simulink model "emso3"  (Simulink 7.1)
settings: Solver=VariableStepDiscrete  StartTime=0.0  StopTime=5  RelTol=1e-3
settings Model: Creator=lades  LastModifiedBy=Administrator
settings DataIOCC: ExternalInput=Az
settings DebuggingCC: SolverPrmCheckMsg=none

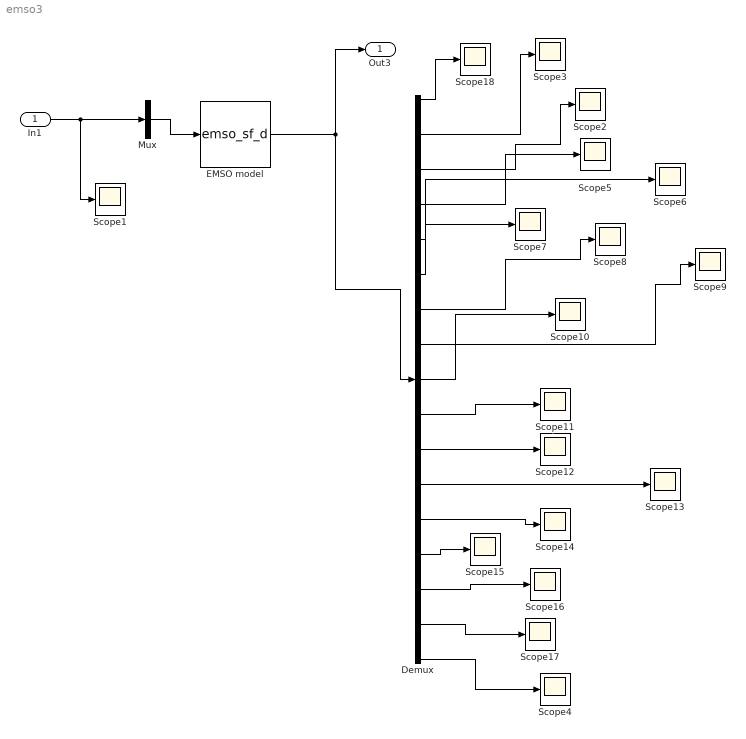
== system emso3 ==
  In1 : Inport  OutDataType=sfix(16)  OutScaling=2^0
  Demux : Demux  Outputs=17
  EMSO model : S-Function  FunctionName=emso_sf_d  Parameters='Diesel_Blend3.ems',6,17,10  EnableBusSupport=off
  Mux : Mux  Inputs=1
  Scope{1..18} (18 alike) : Scope
      Scope1 settings: TimeRange=2  YMin=4.008258966500001  YMax=4.008258969500001
      Scope10 settings: TimeRange=5  YMin=0  YMax=45  SaveName=ScopeData9
      Scope11 settings: TimeRange=5  YMin=0  YMax=45  SaveName=ScopeData10
      Scope12 settings: TimeRange=5  YMin=0  YMax=45  SaveName=ScopeData11
      Scope13 settings: TimeRange=5  YMin=0  YMax=45  SaveName=ScopeData12
      Scope14 settings: TimeRange=5  YMin=0  YMax=45  SaveName=ScopeData13
      Scope15 settings: TimeRange=5  YMin=0  YMax=45  SaveName=ScopeData14
      Scope16 settings: TimeRange=5  YMin=0  YMax=45  SaveName=ScopeData15
      Scope17 settings: TimeRange=5  YMin=0  YMax=45  SaveName=ScopeData16
      Scope18 settings: TimeRange=5  YMin=0  YMax=45  SaveName=ScopeData17
      Scope2 settings: TimeRange=5  YMin=0  YMax=45
      Scope3 settings: TimeRange=5  YMin=0  YMax=45  SaveName=ScopeData2
      Scope4 settings: TimeRange=5  YMin=0  YMax=45  SaveName=ScopeData3
      Scope5 settings: TimeRange=5  YMin=0  YMax=45  SaveName=ScopeData4
      Scope6 settings: TimeRange=5  YMin=0  YMax=45  SaveName=ScopeData5
      Scope7 settings: TimeRange=5  YMin=0  YMax=45  SaveName=ScopeData6
      Scope8 settings: TimeRange=5  YMin=0  YMax=45  SaveName=ScopeData7
      Scope9 settings: TimeRange=5  YMin=0  YMax=45  SaveName=ScopeData8
  Out3 : Outport  OutDataType=sfix(16)  OutScaling=2^0
  wires:
  EMSO model/1 -> Demux/1, Out3/1
  Mux/1 -> EMSO model/1
  In1/1 -> Mux/1, Scope1/1
  Demux/3 -> Scope2/1
  Demux/2 -> Scope3/1
  Demux/4 -> Scope5/1
  Demux/5 -> Scope6/1
  Demux/6 -> Scope7/1
  Demux/7 -> Scope8/1
  Demux/8 -> Scope9/1
  Demux/9 -> Scope10/1
  Demux/10 -> Scope11/1
  Demux/11 -> Scope12/1
  Demux/12 -> Scope13/1
  Demux/13 -> Scope14/1
  Demux/14 -> Scope15/1
  Demux/15 -> Scope16/1
  Demux/16 -> Scope17/1
  Demux/17 -> Scope4/1
  Demux/1 -> Scope18/1
